simulink model "SistemaP4"  (R2026b)
settings: Solver=ode15s  StopTime=10  MaxStep=1e-2
libraries: fl_lib x10, nesl_utility x6, ee_lib x4, slpidlib x1
settings Model: Creator=Maibr  LastModifiedBy=Maibr
settings DataIOCC: DSMLogging=off  ReturnWorkspaceOutputs=off  SaveOutput=off  SignalLogging=off  TimeSaveName=t
settings DebuggingCC: AlgebraicLoopMsg=none  ArtificialAlgebraicLoopMsg=none  BusObjectLabelMismatch=none  MaxConsecutiveZCsMsg=none  OperatingPointInterfaceChecksumMismatchMsg=none  RootOutportRequireBusObject=none
settings RTWCC: DLArmComputeVersion=19.05
settings SimscapeCC: SimscapeUseEnergyAccounting=off

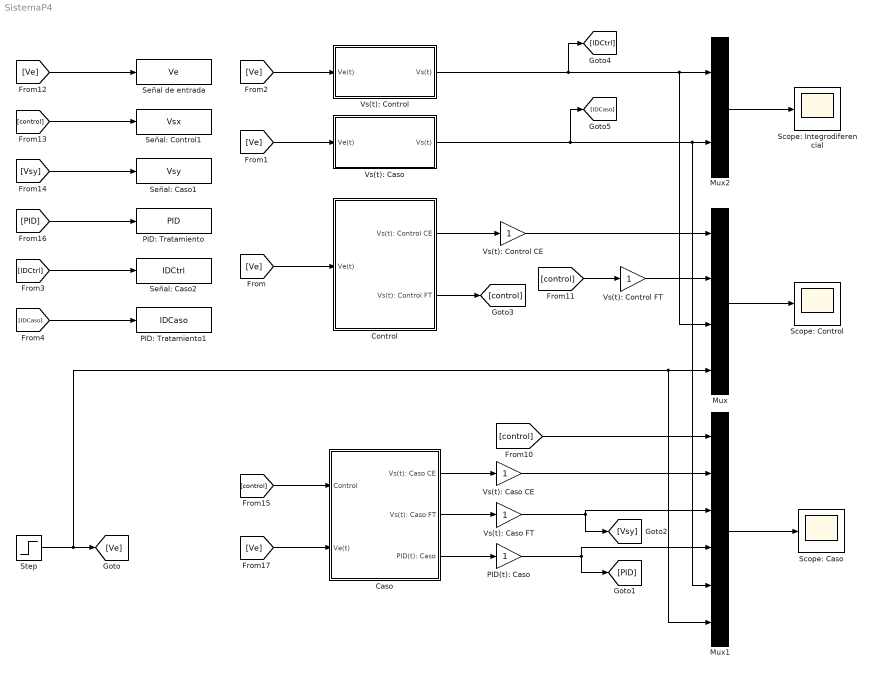
== system SistemaP4 ==
  Caso : Subsystem
  Control : Subsystem
  Mux : Mux
  Mux1 : Mux  Inputs=6
  Mux2 : Mux  Inputs=2
  PID(t): Caso : Gain
  PID: Tratamiento : ToWorkspace  VariableName=PID  SampleTime=-1
  PID: Tratamiento1 : ToWorkspace  VariableName=IDCaso  SampleTime=-1
  Scope: Caso : Scope
      settings: ActiveDisplayYMinimum=-0.18664332863597644  ActiveDisplayYMaximum=1.6958864463640242
  Scope: Control : Scope
      settings: ActiveDisplayYMinimum=-0.065791258378066431  ActiveDisplayYMaximum=1.4829706463838381  DataLoggingVariableName=ScopeData2
  Scope: Integrodiferencial : Scope
      settings: ActiveDisplayYMinimum=-0.68373143834419858  ActiveDisplayYMaximum=1.221217065782169
  Señal de entrada : ToWorkspace  VariableName=Ve  SampleTime=-1
  Señal: Caso1 : ToWorkspace  VariableName=Vsy  SampleTime=-1
  Señal: Caso2 : ToWorkspace  VariableName=IDCtrl  SampleTime=-1
  Señal: Control1 : ToWorkspace  VariableName=Vsx  SampleTime=-1
  Step : Step  InitialValue=1  SampleTime=0
  Vs(t): Caso : Subsystem
  Vs(t): Caso CE : Gain
  Vs(t): Caso FT : Gain
  Vs(t): Control : Subsystem
  Vs(t): Control CE : Gain
  Vs(t): Control FT : Gain
  wires:
  [control] -> Mux1/1
  [PID] -> PID: Tratamiento/1
  Caso/2(Vs(t): Caso FT) -> Vs(t): Caso FT/1
  Vs(t): Caso FT/1 -> [Vsy], Mux1/3
  Vs(t): Control CE/1 -> Mux/1
  [Ve] -> Señal de entrada/1
  Vs(t): Caso CE/1 -> Mux1/2
  [Vsy] -> Señal: Caso1/1
  Control/1(Vs(t): Control CE) -> Vs(t): Control CE/1
  Caso/3(PID(t): Caso) -> PID(t): Caso/1
  Step/1 -> Mux1/6, Mux/4, [Ve]
  PID(t): Caso/1 -> [PID], Mux1/4
  [control] -> Caso/1(Control)
  [Ve] -> Control/1(Ve(t))
  Mux/1 -> Scope: Control/1
  Mux1/1 -> Scope: Caso/1
  [Ve] -> Caso/2(Ve(t))
  [control] -> Señal: Control1/1
  Vs(t): Control FT/1 -> Mux/2
  [control] -> Vs(t): Control FT/1
  Caso/1(Vs(t): Caso CE) -> Vs(t): Caso CE/1
  Control/2(Vs(t): Control FT) -> [control]
  [Ve] -> Vs(t): Caso/1(Ve(t))
  [Ve] -> Vs(t): Control/1(Ve(t))
  Vs(t): Caso/1(Vs(t)) -> [IDCaso], Mux1/5, Mux2/2
  Vs(t): Control/1(Vs(t)) -> [IDCtrl], Mux/3, Mux2/1
  Mux2/1 -> Scope: Integrodiferencial/1
  [IDCtrl] -> Señal: Caso2/1
  [IDCaso] -> PID: Tratamiento1/1

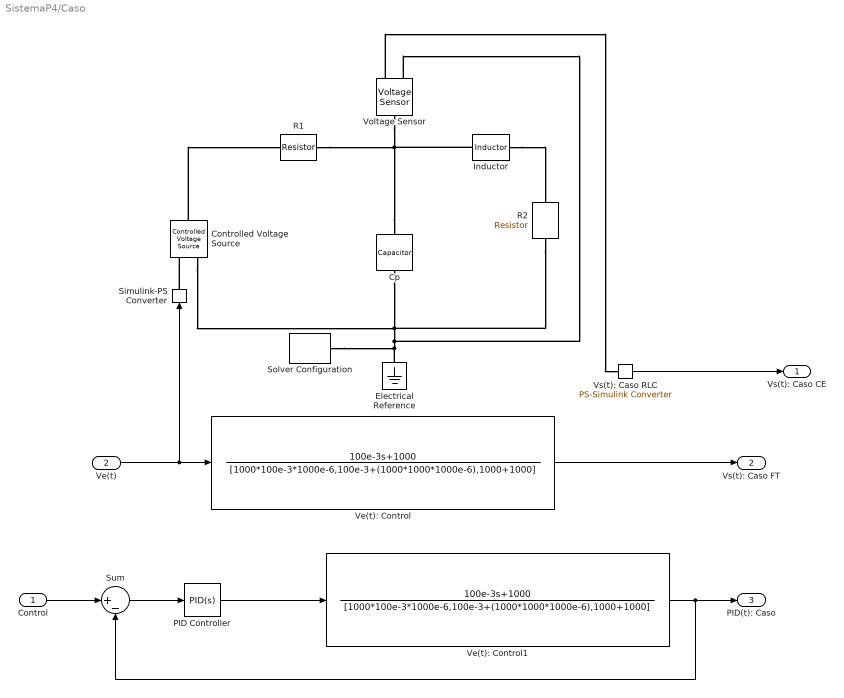
== system SistemaP4/Caso ==
  Control : Inport
  Ve(t) : Inport  Port=2
  Controlled Voltage Source : fl_lib/Electrical/Electrical Sources/Controlled Voltage Source
  Cp : fl_lib/Electrical/Electrical Elements/Capacitor  c=1000e-6 F  r=1e-6 Ohm  g=0 1/Ohm  i_specify=off  i_priority=None  i=0 A  i_nominal_specify=off  i_nominal_value=1  i_nominal_unit=A  v_specify=off  v_priority=None  v=0 V  v_nominal_specify=off  v_nominal_value=1  v_nominal_unit=V  vc_specify=off  vc_priority=High  vc=0 V  vc_nominal_specify=off  vc_nominal_value=1  vc_nominal_unit=V
  Electrical Reference : fl_lib/Electrical/Electrical Elements/Electrical Reference
  Inductor : fl_lib/Electrical/Electrical Elements/Inductor  l=100 mH  r=0 Ohm  g=1e-9 1/Ohm  i_specify=off  i_priority=None  i=0 A  i_nominal_specify=off  i_nominal_value=1  i_nominal_unit=A  v_specify=off  v_priority=None  v=0 V  v_nominal_specify=off  v_nominal_value=1  v_nominal_unit=V  i_L_specify=off  i_L_priority=High  i_L=0 A  i_L_nominal_specify=off  i_L_nominal_value=1  i_L_nominal_unit=A
  PID Controller : slpidlib/PID Controller  Controller=PID  Form=Parallel  TimeDomain=Continuous-time  UseExternalTs=off  SampleTime=-1  IntegratorMethod=Forward Euler  FilterMethod=Forward Euler  ControllerParametersSource=internal  P=1289.29645872171  I=307839.683737193  UseKiTs=off  D=0.179671301047242  UseExternalDerivativeSource=off  N=4928.14063077163  UseFilter=on  TunerSelectOption=Transfer Function Based (PID Tuner App)  InitialConditionSource=internal  InitialConditionForIntegrator=0  InitialConditionForFilter=0  DifferentiatorICPrevScaledInput=0  ExternalReset=none  TrackingMode=off  Kt=1  LimitOutput=off  SatLimitsSource=internal  UpperSaturationLimit=inf  LowerSaturationLimit=-inf  LinearizeAsGain=on  AntiWindupMode=none  Kb=1  LimitIntegrator=off  UpperIntegratorSaturationLimit=inf  LowerIntegratorSaturationLimit=-inf  POutMin=[]  POutMax=[]  IOutMin=[]  IOutMax=[]  DOutMin=[]  DOutMax=[]  NOutMin=[]  NOutMax=[]  SumOutMin=[]  SumOutMax=[]  SaturationOutMin=[]  SaturationOutMax=[]  PParamMin=[]  PParamMax=[]  IParamMin=[]  IParamMax=[]  DParamMin=[]  DParamMax=[]  NParamMin=[]  NParamMax=[]  KbParamMin=[]  KbParamMax=[]  KtParamMin=[]  KtParamMax=[]  KbOutMin=[]  KbOutMax=[]  KtOutMin=[]  KtOutMax=[]  IntegratorOutMin=[]  IntegratorOutMax=[]  FilterOutMin=[]  FilterOutMax=[]  SumI1OutMin=[]  SumI1OutMax=[]  SumI2OutMin=[]  SumI2OutMax=[]  SumI3OutMin=[]  SumI3OutMax=[]  SumI4OutMin=[]  SumI4OutMax=[]  SumDOutMin=[]  SumDOutMax=[]  DifferentiatorOutMin=[]  DifferentiatorOutMax=[]  FilterDiffOutCoefMin=[]  FilterDiffOutCoefMax=[]  ReciprocalOutMin=[]  ReciprocalOutMax=[]  SumDenOutMin=[]  SumDenOutMax=[]  SumNumOutMin=[]  SumNumOutMax=[]  DivideOutMin=[]  DivideOutMax=[]  UdiffTsProdOutMin=[]  UdiffTsProdOutMax=[]  NTsProdOutMin=[]  NTsProdOutMax=[]  UintegralTsProdOutMin=[]  UintegralTsProdOutMax=[]  UngainTsProdOutMin=[]  UngainTsProdOutMax=[]  ClampingZeroOutDataTypeStr=Inherit: Inherit via back propagation  ClampingZeroOutMin=[]  ClampingZeroOutMax=[]  FilterDenConstantOutDataTypeStr=Inherit: Inherit via back propagation  FilterDenConstantOutMin=[]  FilterDenConstantOutMax=[]  PCopyOutDataTypeStr=Inherit: Inherit via back propagation  PCopyOutMin=[]  PCopyOutMax=[]  NCopyOutDataTypeStr=Inherit: Inherit via back propagation  NCopyOutMin=[]  NCopyOutMax=[]  IntegratorContinuousStateAttributes=''  IntegratorStateMustResolveToSignalObject=off  IntegratorRTWStateStorageClass=Auto  FilterContinuousStateAttributes=''  FilterStateMustResolveToSignalObject=off  FilterRTWStateStorageClass=Auto  ParallelPVariant=InternalParameters  IdealPVariant=Disabled  IVariant=InternalParameters  DVariant=InternalParameters  IntegratorVariant=Continuous  SatVariant=Disabled  AWVariant=Passthrough  PCopyVariant=Disabled  TRVariant=Disabled  FdbkBlocksVariant=Forward  IdealPFdbkVariant=Disabled  SatFdbkVariant=Disabled  DerivativeFilterVariant=ContFilter  NVariant=InternalParameters  NCopyVariant=Disabled  FilterICVariant=InternalICsFilter  IntegratorICVariant=InternalICs  ExternalResetVariant=Disabled  TRSumVariant=Passthrough  SumFdbkVariant=Disabled  SumVariant=Sum_PID  TsampFilterVariant=InternalTs  TsampNgainVariant=Passthrough  TsampIntegralVariant=Disabled_SignalSpec  ExternalSaturationOutDataTypeStr=Inherit: Same as second input  DerivativeSourceVariant=ErrorSignal  PreIntVariant=InternalPreInt
  R1 : ee_lib/Passive/Resistor  R=1000 Ohm  enable_R_tol=0  R_tol=5  tol_distribution=1  nSigma=4  enable_operating_limits=0  operating_limit_action=2  power_rating=1 W  max_working_voltage=100 V  noise_mode=0  Tdevice=25 degC  sample_time=1e-3 s  repeatability=1  user_seed=0  auto_seed=3499211588  power_derating_T1=70 degC  power_derating_T2=155 degC  operating_temperature_range_vec=[-50, 150] degC  alpha=3.93e-3 1/K  Tmeas=25 degC  thermal_mass=100 J/K  temperature_specify=off  temperature_priority=High  temperature=298.15 K  temperature_nominal_specify=off  temperature_nominal_value=1  temperature_nominal_unit=K
  R2 : ee_lib/Passive/Resistor  R=1000 Ohm  enable_R_tol=0  R_tol=5  tol_distribution=1  nSigma=4  enable_operating_limits=0  operating_limit_action=2  power_rating=1 W  max_working_voltage=100 V  noise_mode=0  Tdevice=25 degC  sample_time=1e-3 s  repeatability=1  user_seed=0  auto_seed=3890346746  power_derating_T1=70 degC  power_derating_T2=155 degC  operating_temperature_range_vec=[-50, 150] degC  alpha=3.93e-3 1/K  Tmeas=25 degC  thermal_mass=100 J/K  temperature_specify=off  temperature_priority=High  temperature=298.15 K  temperature_nominal_specify=off  temperature_nominal_value=1  temperature_nominal_unit=K
  Simulink-PS Converter : nesl_utility/Simulink-PS Converter  PhysicalDomain=network_engine_domain  SubClassName=ps_input  LeftPortType=input  RightPortType=output  PseudoPeriodic=off  Frequencies=[]  NoiseDistribution=none  NoiseParameters=[]  Unit=1  AffineConversion=off  FilteringAndDerivatives=provide  SimscapeFilterOrder=1  InputFilterTimeConstant=0.001  UdotUserProvided=0
  Solver Configuration : nesl_utility/Solver Configuration  PhysicalDomain=network_engine_domain  SubClassName=solver  LeftPortType=input  RightPortType=generic  Tones=[]  Harmonics=[]  SimulateNoise=off  Profile=off  UseLocalSampling=off  EnableSwitchedLinearOptims=on  FrequencyDomain=off  UseCCode=off  RelTol=0.001  AbsTol=1e-06  MinStep=1e-09  ToWorkspace=off  RevertToSquareIcSolve=off  NumHomotopyIterations=100  PhasorMode=off  PhasorModeNumHarmonics=1  ConsistencySolver=NEWTON_FTOL  CanonicalOrdering=UNORDERED  OptimizeIntermediates=UNOPTIMIZED  MulticoreSolverChoice=BACKWARD_EULER  IndexReductionMethod=DerivativeReplacement  DoDC=off  ResidualTolerance=1e-09  ConsistencyTolSource=GLOBAL  ConsistencyAbsTol=0.001  ConsistencyRelTol=0.001  ConsistencyTolFactor=0.001  UseLocalSolver=off  LocalSolverChoice=NE_BACKWARD_EULER_ADVANCER  ResolveIndetEquations=on  FunctionEvalNumThread=1  LocalSolverSampleTime=0.001  DoFixedCost=off  MaxNonlinIter=3  MaxModeIter=2  ComputeImpulses=off  ImpulseIterations=2  LinearAlgebra=auto  LinearAlgebraNumThread=0  EquationFormulation=NE_TIME_EF  DelaysMemoryBudget=1024  AutomaticFiltering=on  FilteringTimeConstant=0.001  PartitionStorageMethod=AS_NEEDED  PartitionMemoryBudget=1024  PartitionMethod=BALANCED  MultibodyUseLocalSolver=off  MultibodyLocalSolverChoice=ODE1  MultibodyLocalSolverSampleTime=0.001
  Sum : Sum  Inputs=|+-
  Ve(t): Control : TransferFcn  Numerator=[100e-3,1000]  Denominator=[1000*100e-3*1000e-6,100e-3+(1000*1000*1000e-6),1000+1000]
  Ve(t): Control1 : TransferFcn  Numerator=[100e-3,1000]  Denominator=[1000*100e-3*1000e-6,100e-3+(1000*1000*1000e-6),1000+1000]
  Voltage Sensor : fl_lib/Electrical/Electrical Sensors/Voltage Sensor
  "Vs(t): Caso RLC " : nesl_utility/PS-Simulink Converter  PhysicalDomain=network_engine_domain  SubClassName=ps_output  LeftPortType=input  RightPortType=output  PseudoPeriodic=off  Frequencies=[]  VectorFormat=1-D array  Unit=inherit  AffineConversion=off
  Vs(t): Caso CE : Outport
  Vs(t): Caso FT : Outport  Port=2
  PID(t): Caso : Outport  Port=3
  wires:
  Sum/1 -> PID Controller/1
  PID Controller/1 -> Ve(t): Control1/1
  Control/1 -> Sum/1
  Ve(t): Control/1 -> Vs(t): Caso FT/1
  Ve(t): Control1/1 -> Sum/2, PID(t): Caso/1
  "Vs(t): Caso RLC "/1 -> Vs(t): Caso CE/1
  Ve(t)/1 -> Simulink-PS Converter/1, Ve(t): Control/1
  connections:
  Cp/RConn1 -- R2/LConn1 -- Controlled Voltage Source/RConn2 -- Voltage Sensor/RConn2 -- Electrical Reference/LConn1 -- Solver Configuration/RConn1
  Cp/LConn1 -- Voltage Sensor/LConn1 -- R1/LConn1 -- Inductor/LConn1
  Voltage Sensor/RConn1 -- "Vs(t): Caso RLC "/LConn1
  Controlled Voltage Source/LConn1 -- R1/RConn1
  Simulink-PS Converter/RConn1 -- Controlled Voltage Source/RConn1
  Inductor/RConn1 -- R2/RConn1

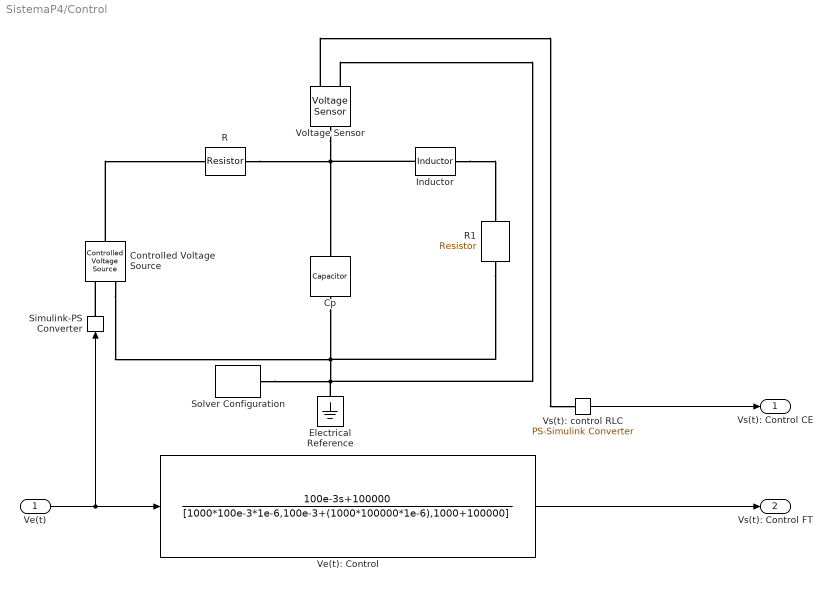
== system SistemaP4/Control ==
  Ve(t) : Inport
  Controlled Voltage Source : fl_lib/Electrical/Electrical Sources/Controlled Voltage Source
  Cp : fl_lib/Electrical/Electrical Elements/Capacitor  c=1e-6 F  r=1e-6 Ohm  g=0 1/Ohm  i_specify=off  i_priority=None  i=0 A  i_nominal_specify=off  i_nominal_value=1  i_nominal_unit=A  v_specify=off  v_priority=None  v=0 V  v_nominal_specify=off  v_nominal_value=1  v_nominal_unit=V  vc_specify=off  vc_priority=High  vc=0 V  vc_nominal_specify=off  vc_nominal_value=1  vc_nominal_unit=V
  Electrical Reference : fl_lib/Electrical/Electrical Elements/Electrical Reference
  Inductor : fl_lib/Electrical/Electrical Elements/Inductor  l=100 mH  r=0 Ohm  g=1e-9 1/Ohm  i_specify=off  i_priority=None  i=0 A  i_nominal_specify=off  i_nominal_value=1  i_nominal_unit=A  v_specify=off  v_priority=None  v=0 V  v_nominal_specify=off  v_nominal_value=1  v_nominal_unit=V  i_L_specify=off  i_L_priority=High  i_L=0 A  i_L_nominal_specify=off  i_L_nominal_value=1  i_L_nominal_unit=A
  R : ee_lib/Passive/Resistor  R=1000 Ohm  enable_R_tol=0  R_tol=5  tol_distribution=1  nSigma=4  enable_operating_limits=0  operating_limit_action=2  power_rating=1 W  max_working_voltage=100 V  noise_mode=0  Tdevice=25 degC  sample_time=1e-3 s  repeatability=1  user_seed=0  auto_seed=545404223  power_derating_T1=70 degC  power_derating_T2=155 degC  operating_temperature_range_vec=[-50, 150] degC  alpha=3.93e-3 1/K  Tmeas=25 degC  thermal_mass=100 J/K  temperature_specify=off  temperature_priority=High  temperature=298.15 K  temperature_nominal_specify=off  temperature_nominal_value=1  temperature_nominal_unit=K
  R1 : ee_lib/Passive/Resistor  R=100000 Ohm  enable_R_tol=0  R_tol=5  tol_distribution=1  nSigma=4  enable_operating_limits=0  operating_limit_action=2  power_rating=1 W  max_working_voltage=100 V  noise_mode=0  Tdevice=25 degC  sample_time=1e-3 s  repeatability=1  user_seed=0  auto_seed=3922919431  power_derating_T1=70 degC  power_derating_T2=155 degC  operating_temperature_range_vec=[-50, 150] degC  alpha=3.93e-3 1/K  Tmeas=25 degC  thermal_mass=100 J/K  temperature_specify=off  temperature_priority=High  temperature=298.15 K  temperature_nominal_specify=off  temperature_nominal_value=1  temperature_nominal_unit=K
  Simulink-PS Converter : nesl_utility/Simulink-PS Converter  PhysicalDomain=network_engine_domain  SubClassName=ps_input  LeftPortType=input  RightPortType=output  PseudoPeriodic=off  Frequencies=[]  NoiseDistribution=none  NoiseParameters=[]  Unit=1  AffineConversion=off  FilteringAndDerivatives=provide  SimscapeFilterOrder=1  InputFilterTimeConstant=0.001  UdotUserProvided=0
  Solver Configuration : nesl_utility/Solver Configuration  PhysicalDomain=network_engine_domain  SubClassName=solver  LeftPortType=input  RightPortType=generic  Tones=[]  Harmonics=[]  SimulateNoise=off  Profile=off  UseLocalSampling=off  EnableSwitchedLinearOptims=on  FrequencyDomain=off  UseCCode=off  RelTol=0.001  AbsTol=1e-06  MinStep=1e-09  ToWorkspace=off  RevertToSquareIcSolve=off  NumHomotopyIterations=100  PhasorMode=off  PhasorModeNumHarmonics=1  ConsistencySolver=NEWTON_FTOL  CanonicalOrdering=UNORDERED  OptimizeIntermediates=UNOPTIMIZED  MulticoreSolverChoice=BACKWARD_EULER  IndexReductionMethod=DerivativeReplacement  DoDC=off  ResidualTolerance=1e-09  ConsistencyTolSource=GLOBAL  ConsistencyAbsTol=0.001  ConsistencyRelTol=0.001  ConsistencyTolFactor=0.001  UseLocalSolver=off  LocalSolverChoice=NE_BACKWARD_EULER_ADVANCER  ResolveIndetEquations=on  FunctionEvalNumThread=1  LocalSolverSampleTime=0.001  DoFixedCost=off  MaxNonlinIter=3  MaxModeIter=2  ComputeImpulses=off  ImpulseIterations=2  LinearAlgebra=auto  LinearAlgebraNumThread=0  EquationFormulation=NE_TIME_EF  DelaysMemoryBudget=1024  AutomaticFiltering=on  FilteringTimeConstant=0.001  PartitionStorageMethod=AS_NEEDED  PartitionMemoryBudget=1024  PartitionMethod=BALANCED  MultibodyUseLocalSolver=off  MultibodyLocalSolverChoice=ODE1  MultibodyLocalSolverSampleTime=0.001
  Ve(t): Control : TransferFcn  Numerator=[100e-3,100000]  Denominator=[1000*100e-3*1e-6,100e-3+(1000*100000*1e-6),1000+100000]
  Voltage Sensor : fl_lib/Electrical/Electrical Sensors/Voltage Sensor
  "Vs(t): control RLC " : nesl_utility/PS-Simulink Converter  PhysicalDomain=network_engine_domain  SubClassName=ps_output  LeftPortType=input  RightPortType=output  PseudoPeriodic=off  Frequencies=[]  VectorFormat=1-D array  Unit=inherit  AffineConversion=off
  Vs(t): Control CE : Outport
  Vs(t): Control FT : Outport  Port=2
  wires:
  "Vs(t): control RLC "/1 -> Vs(t): Control CE/1
  Ve(t): Control/1 -> Vs(t): Control FT/1
  Ve(t)/1 -> Simulink-PS Converter/1, Ve(t): Control/1
  connections:
  Electrical Reference/LConn1 -- Solver Configuration/RConn1 -- Voltage Sensor/RConn2 -- R1/LConn1 -- Controlled Voltage Source/RConn2 -- Cp/RConn1
  Simulink-PS Converter/RConn1 -- Controlled Voltage Source/RConn1
  Controlled Voltage Source/LConn1 -- R/RConn1
  R/LConn1 -- Voltage Sensor/LConn1 -- Inductor/LConn1 -- Cp/LConn1
  Inductor/RConn1 -- R1/RConn1
  Voltage Sensor/RConn1 -- "Vs(t): control RLC "/LConn1

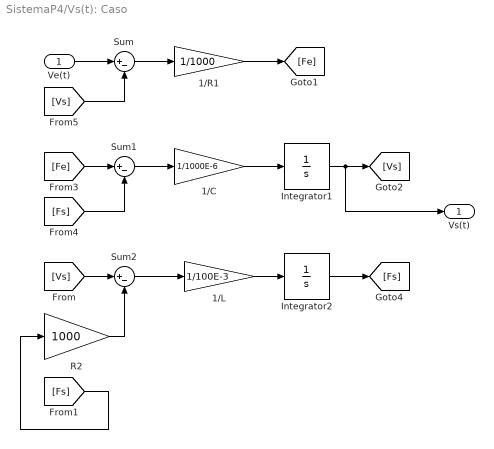
== system SistemaP4/Vs(t): Caso ==
  Ve(t) : Inport
  1/C : Gain  Gain=1/1000E-6
  1/L : Gain  Gain=1/100E-3
  1/R1 : Gain  Gain=1/1000
  Integrator1 : Integrator
  Integrator2 : Integrator
  R2 : Gain  Gain=1000
  Sum : Sum  Inputs=|+-
  Sum1 : Sum  Inputs=|+-
  Sum2 : Sum  Inputs=|+-
  Vs(t) : Outport
  wires:
  Ve(t)/1 -> Sum/1
  Sum/1 -> 1/R1/1
  [Vs] -> Sum/2
  1/R1/1 -> [Fe]
  [Fe] -> Sum1/1
  1/C/1 -> Integrator1/1
  Integrator1/1 -> Vs(t)/1, [Vs]
  Sum1/1 -> 1/C/1
  [Fs] -> Sum1/2
  [Vs] -> Sum2/1
  Sum2/1 -> 1/L/1
  1/L/1 -> Integrator2/1
  Integrator2/1 -> [Fs]
  [Fs] -> R2/1
  R2/1 -> Sum2/2

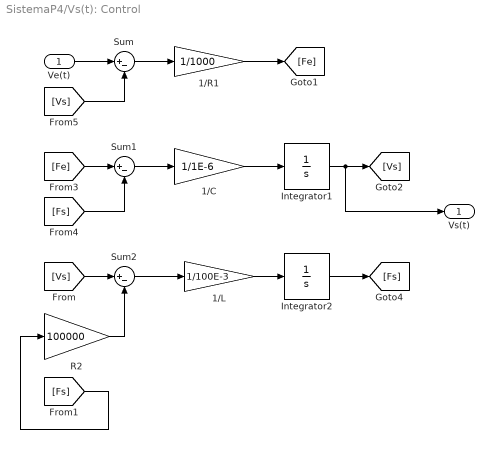
== system SistemaP4/Vs(t): Control ==
  Ve(t) : Inport
  1/C : Gain  Gain=1/1E-6
  1/L : Gain  Gain=1/100E-3
  1/R1 : Gain  Gain=1/1000
  Integrator1 : Integrator
  Integrator2 : Integrator
  R2 : Gain  Gain=100000
  Sum : Sum  Inputs=|+-
  Sum1 : Sum  Inputs=|+-
  Sum2 : Sum  Inputs=|+-
  Vs(t) : Outport
  wires:
  Ve(t)/1 -> Sum/1
  Sum/1 -> 1/R1/1
  [Vs] -> Sum/2
  1/R1/1 -> [Fe]
  [Fe] -> Sum1/1
  1/C/1 -> Integrator1/1
  Integrator1/1 -> Vs(t)/1, [Vs]
  Sum1/1 -> 1/C/1
  [Fs] -> Sum1/2
  [Vs] -> Sum2/1
  Sum2/1 -> 1/L/1
  1/L/1 -> Integrator2/1
  Integrator2/1 -> [Fs]
  [Fs] -> R2/1
  R2/1 -> Sum2/2
